simulink model "Generation"  (R2021b)
settings: Solver=FixedStepAuto  StartTime=0.0  StopTime=10.0  RelTol=1e-3
settings Model: Creator=PRO  LastModifiedBy=PRO
settings OptimizationCC: DefaultParameterBehavior=Inlined  EnhancedBackFolding=on  PassReuseOutputArgsAs=Individual arguments  ZeroExternalMemoryAtStartup=off  ZeroInternalMemoryAtStartup=off  OptimizeBlockOrder=speed  DifferentSizesBufferReuse=on  OptimizationCustomize=off  EfficientTunableParamExpr=on
settings DebuggingCC: ParameterTunabilityLossMsg=error
settings SFSimCC: MATLABDynamicMemAlloc=off
settings RTWCC: Description=Embedded Coder  SystemTargetFile=ert.tlc  TemplateMakefile=ert_default_tmf
settings CodeAppCC: ForceParamTrailComments=on  IgnoreCustomStorageClasses=off  OperatorAnnotations=on  SimulinkDataObjDesc=on  SFDataObjDesc=on  CustomSymbolStrType=$R$N$M_T  InsertBlockDesc=on
settings ERTTargetCC: TargetLangStandard=C99 (ISO)  GenerateSampleERTMain=on  SupportComplex=off  SupportContinuousTime=on  InlinedParameterPlacement=NonHierarchical  ERTCustomFileTemplate=example_file_process.tlc

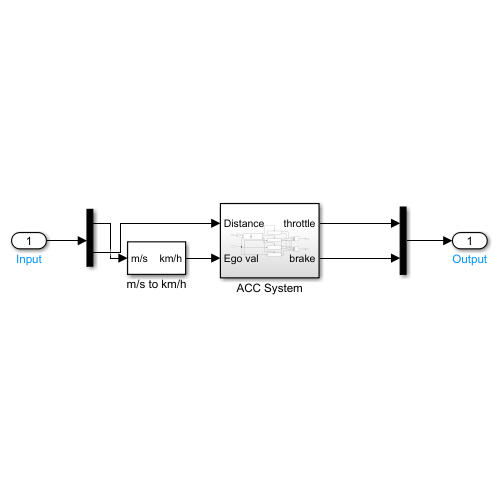
[thumbnail: Simulink's stored preview of the top-level diagram]
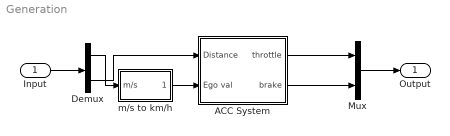
== system Generation ==
  Input : Inport
  ACC System : Subsystem
  Demux : Demux  Outputs=2
  Mux : Mux  Inputs=2
  m/s to km/h : Subsystem
  Output : Outport
  wires:
  Mux/1 -> Output/1
  Input/1 -> Demux/1
  Demux/1 -> m/s to km/h/1(m/s)
  Demux/2 -> ACC System/1(Distance)
  m/s to km/h/1(km/h) -> ACC System/2(Ego val)
  ACC System/1(throttle) -> Mux/1
  ACC System/2(brake) -> Mux/2

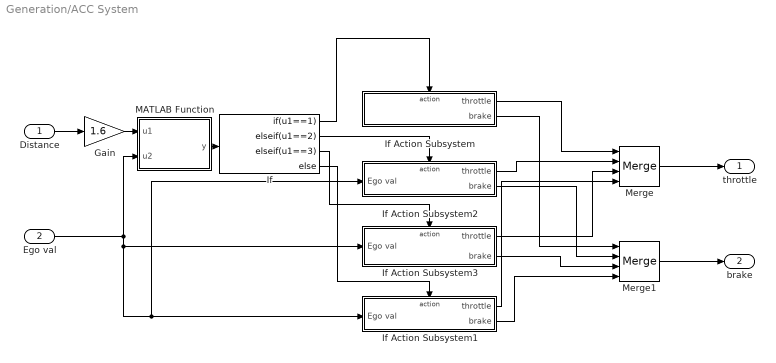
== system Generation/ACC System ==
  Distance : Inport
  Ego val : Inport  Port=2
  Gain : Gain  Gain=1.6
  If : If  IfExpression=u1==1  ElseIfExpressions=u1==2, u1==3
  If Action Subsystem : Subsystem  TreatAsAtomicUnit=on
  If Action Subsystem1 : Subsystem  TreatAsAtomicUnit=on
  If Action Subsystem2 : Subsystem  TreatAsAtomicUnit=on
  If Action Subsystem3 : Subsystem  TreatAsAtomicUnit=on
  MATLAB Function : MATLAB Function  TreatAsAtomicUnit=on
  Merge : Merge  Inputs=4
  Merge1 : Merge  Inputs=4
  throttle : Outport
  brake : Outport  Port=2
  wires:
  Ego val/1 -> MATLAB Function/2(u2), If Action Subsystem2/1(Ego val), If Action Subsystem1/1(Ego val), If Action Subsystem3/1(Ego val)
  If/1 -> If Action Subsystem/Action
  If/4 -> If Action Subsystem1/Action
  If Action Subsystem1/1(throttle) -> Merge/4
  If Action Subsystem/2(brake) -> Merge1/1
  If Action Subsystem1/2(brake) -> Merge1/4
  MATLAB Function/1(y) -> If/1
  Distance/1 -> Gain/1
  Gain/1 -> MATLAB Function/1(u1)
  If/2 -> If Action Subsystem2/Action
  If Action Subsystem2/1(throttle) -> Merge/2
  If Action Subsystem2/2(brake) -> Merge1/2
  If/3 -> If Action Subsystem3/Action
  If Action Subsystem3/1(throttle) -> Merge/3
  If Action Subsystem3/2(brake) -> Merge1/3
  Merge1/1 -> brake/1
  Merge/1 -> throttle/1
  If Action Subsystem/1(throttle) -> Merge/1

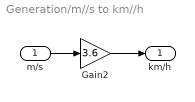
== system Generation/m//s to km//h ==
  m/s : Inport
  Gain2 : Gain  Gain=3.6
  km/h : Outport
  wires:
  Gain2/1 -> km/h/1
  m/s/1 -> Gain2/1

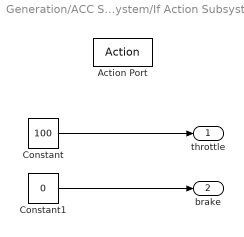
== system Generation/ACC System/If Action Subsystem ==
  Action Port : ActionPort  ActionPortLabel=if(u1==1)
  Constant : Constant  Value=100
  Constant1 : Constant  Value=0
  throttle : Outport
  brake : Outport  Port=2
  wires:
  Constant1/1 -> brake/1
  Constant/1 -> throttle/1

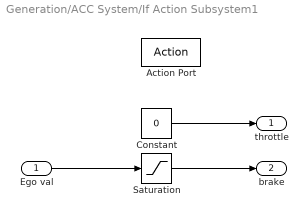
== system Generation/ACC System/If Action Subsystem1 ==
  Ego val : Inport
  Action Port : ActionPort  ActionPortLabel=else
  Constant : Constant  Value=0
  Saturation : Saturate  UpperLimit=40  LowerLimit=0  OutDataTypeStr=double
  throttle : Outport
  brake : Outport  Port=2
  wires:
  Constant/1 -> throttle/1
  Ego val/1 -> Saturation/1
  Saturation/1 -> brake/1

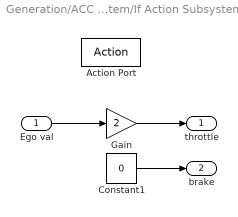
== system Generation/ACC System/If Action Subsystem2 ==
  Ego val : Inport
  Action Port : ActionPort  ActionPortLabel=elseif(u1==2)
  Constant1 : Constant  Value=0
  Gain : Gain  Gain=2  OutDataTypeStr=double
  throttle : Outport
  brake : Outport  Port=2
  wires:
  Gain/1 -> throttle/1
  Constant1/1 -> brake/1
  Ego val/1 -> Gain/1

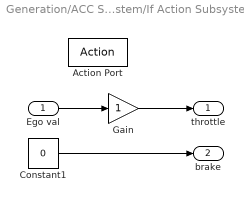
== system Generation/ACC System/If Action Subsystem3 ==
  Ego val : Inport
  Action Port : ActionPort  ActionPortLabel=elseif( u1==3)
  Constant1 : Constant  Value=0
  Gain : Gain  ParamDataTypeStr=double
  throttle : Outport
  brake : Outport  Port=2
  wires:
  Constant1/1 -> brake/1
  Ego val/1 -> Gain/1
  Gain/1 -> throttle/1

== matlab function Generation/ACC System/MATLAB Function ==
  data: u1 input; y output; u2 input
function y = fcn(u1, u2)
    if (u1 > u2) % 뒤 치량이 앞 차량보다 많이 늦을 때
        y = 1; 
    elseif (0.9*u1<u2)&&(u2<1.1*u1) % 두 차량이 안전거리를 유지할 때
        y=2;
    elseif (u1 == 0) % 두 차량이 감지하지 못할 때
        y=3;
    else
        y = 0; % 뒤 차량이 앞 차량보다 빠를 때
    end
end
